simulink model "state_machine"  (R2023b)
settings: Solver=FixedStepDiscrete  StartTime=0.0  StopTime=10.0  FixedStep=0.001  RelTol=1e-3
settings Model: DataDictionary=state_machine.sldd  Creator=admin  LastModifiedBy=admin
settings OptimizationCC: DefaultParameterBehavior=Inlined  EnhancedBackFolding=on  PassReuseOutputArgsAs=Individual arguments  ActiveStateOutputEnumStorageType=uint8  ZeroExternalMemoryAtStartup=off  ZeroInternalMemoryAtStartup=off  EfficientFloat2IntCast=on  OptimizeBlockOrder=speed  DifferentSizesBufferReuse=on  OptimizationCustomize=off  EfficientTunableParamExpr=on
settings DebuggingCC: ParameterTunabilityLossMsg=error
settings HardwareCC: ProdBitPerPointer=32  ProdBitPerSizeT=32  ProdBitPerPtrDiffT=32  ProdLargestAtomicInteger=Long  ProdLargestAtomicFloat=Double  ProdWordSize=32  ProdHWDeviceType=ARM Compatible->ARM Cortex-M
settings SFSimCC: MATLABDynamicMemAlloc=off
settings RTWCC: Description=Embedded Coder  SystemTargetFile=ert.tlc  GenCodeOnly=on  TemplateMakefile=ert_default_tmf  GenerateReport=on  IncludeHyperlinkInReport=on  LaunchReport=on  GenerateTraceInfo=on  GenerateTraceReportSl=on  GenerateTraceReportSf=on  GenerateWebview=on
settings CodeAppCC: ForceParamTrailComments=on  IgnoreCustomStorageClasses=off  OperatorAnnotations=on  SimulinkDataObjDesc=on  SFDataObjDesc=on  InsertBlockDesc=on
settings ERTTargetCC: TargetLangStandard=C99 (ISO)  IncludeMdlTerminateFcn=off  SupportNonFinite=off  SupportComplex=off  RemoveDisableFunc=on  InlinedParameterPlacement=NonHierarchical  ERTCustomFileTemplate=example_file_process.tlc  ERTFilePackagingFormat=CompactWithDataFile

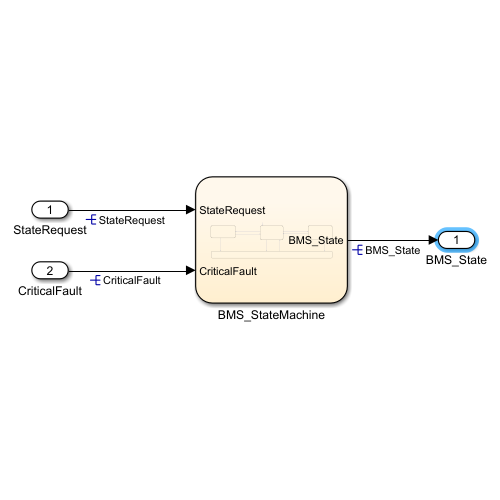
[thumbnail: Simulink's stored preview of the top-level diagram]
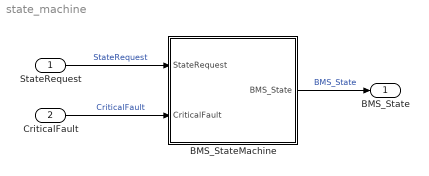
== system state_machine ==
  StateRequest : Inport  OutDataTypeStr=Enum: SRE
  CriticalFault : Inport  Port=2  OutDataTypeStr=boolean
  BMS_StateMachine : Stateflow chart  TreatAsAtomicUnit=on
  BMS_State : Outport  OutDataTypeStr=Enum: BMS_State_Enum
  wires:
  CriticalFault/1 -> BMS_StateMachine/2(CriticalFault)  "CriticalFault"
  StateRequest/1 -> BMS_StateMachine/1(StateRequest)  "StateRequest"
  BMS_StateMachine/1(BMS_State) -> BMS_State/1  "BMS_State"

== stateflow chart state_machine/BMS_StateMachine ==
  state Driving
    en:
    BMS_State = ...
    BMS_State_Enum.BMS_Driving;
  state Standby
    en:
    BMS_State = ...
    BMS_State_Enum.BMS_Standby;
  state Charging
    en:
    BMS_State = ...
    BMS_State_Enum.BMS_Charging;
  state Fault
    en,du:
    BMS_State = BMS_State_Enum.BMS_Fault;
  (default) -> Standby
  Standby -> Charging [order 1] : [StateRequest ==SRE.Charging]
  Standby -> Driving [order 3] : [StateRequest == SRE.Driving]
  Charging -> Standby [order 2] : [StateRequest ~=SRE.Charging]
  Driving -> Standby [order 2] : [StateRequest ~= SRE.Driving]
  Driving -> Fault [order 1] : [CriticalFault]
  Standby -> Fault [order 2] : [CriticalFault]
  Fault -> Standby : [~CriticalFault]
  Charging -> Fault [order 1] : [CriticalFault]
  data: StateRequest input Enum: SRE; BMS_State output Enum: BMS_State_Enum; CriticalFault input boolean
